simulink model "afe_rst_inv_psm_distributed_control_two_delays"  (R2026a)
settings: Solver=ode1be  StopTime=simlength  FixedStep=tc  MaxStep=Tc
values from neighbouring files (symbols this model uses):
  Amplitude_U = 1.16    [grid_fault_generator.m]
  Amplitude_V = Amplitude_U    (= 1.16)    [grid_fault_generator.m]
  Amplitude_W = Amplitude_U    (= 1.16)    [grid_fault_generator.m]
  end_time_LVRT = start_time_LVRT + error_length    [grid_fault_generator.m]
  Igrid_phase_normalization_factor = 270*sqrt(2)    [grid_emulator.m]
  omega_grid_emulator_nom = w_grid    (= 314.159265359)    [grid_emulator.m]
  omega_grid_nom = w_grid    (= 314.159265359)    [grid_emulator.m]
  t_ramp = 20e-3    (= 0.02)    [grid_fault_generator.m]
  ugrid_factor = 1    [grid_emulator.m]
  V_phase_normalization_factor = Vgrid_phase_normalization_factor    [grid_emulator.m]
  Vdc_bez = 1070    [grid_emulator.m]
  Vemu_ref_norm = Vemu_ref * sqrt(2) / V_phase_normalization_factor    [grid_emulator.m]
  vn_eta_pu = 0    [grid_emulator.m]
  vn_xi_pu = 0    [grid_emulator.m]
  vp_xi_pu = 1    [grid_emulator.m]
undefined symbols (not defined in the file or in its folder): Adrso, Aresd, Bresd, CFi, CFu, Cresd, Crso, CTRPIFF_CLIP_RELEASE, dead_time_INV, emf_fb_p, emf_fb_p_ccaller_1, emf_fb_p_ccaller_2, emf_p, emf_p_ccaller_1, emf_p_ccaller_2, fPWM_INV, g0_161Hz, g0_500Hz, g1_161Hz, g1_500Hz, i_grid_neg_eta_lim, i_grid_neg_eta_red_lim, i_grid_neg_xi_lim, i_grid_neg_xi_red_lim, i_grid_pos_eta_lim, i_grid_pos_eta_red_lim, ibez, id_lim, ieta_neg_ref_lim, ieta_pos_ref_lim, iq_lim, ixi_pos_ref_lim, Jm_norm, k_frt_ref, kg, ki_afe, ki_i, ki_id, ki_iq, ki_rc_neg_grid, ki_rc_pos_grid, ki_vs, ki_w, kp_afe, kp_i, kp_id, kp_iq, kp_rc_neg_grid, kp_rc_pos_grid, kp_vs, kp_w, kw, l1, l2, Lalpha_norm, Ld_norm, Ldrso, Lq_norm, Ls_norm, luenberger_l1 ... (+30)
libraries: fl_lib x146, nesl_utility x62, simulink x8, cstblocks_lti x7, sl_discontinuities x3, single_phase_transformer_lib x3, flexshaft_lib x1, permanent_magnet_synchronous_machine x1
(part 10 of 14)

== system afe_rst_inv_psm_distributed_control_two_delays/INV-Modular/inv_leg_u/driver_board_u/motor_vector_control/bemf_observer/bemf_observer_simulink ==
  ialpha_pu : Inport
  ibeta_pu : Inport  Port=2
  ualpha_pu : Inport  Port=3
  ubeta_pu : Inport  Port=4
  Gain : Gain  Gain=psi_m_norm
  Gain1 : Gain  Gain=psi_m_norm
  Trigonometric Function : Trigonometry  Operator=cos
  Trigonometric Function1 : Trigonometry
  double_integrator_observer : Subsystem
  omega_hat_flt : Subsystem
  psi_alpha_hat : Subsystem
  psi_beta_hat : Subsystem
  theta_bemf_hat : Subsystem
  omega_pu_hat : Outport
  theta_hat : Outport  Port=2
  tag scope: psi_r_m_alpha_dbu=global, psi_r_m_beta_dbu=global, theta_bemf_hat_dbu=global
  wires:
  omega_hat_flt/1(omega_hat_flt) -> theta_bemf_hat/3(omega_pu_hat)
  double_integrator_observer/1(omega_pu_hat) -> omega_hat_flt/1(omega_hat), omega_pu_hat/1  "omega_pu_hat"
  double_integrator_observer/2(theta_hat) -> theta_hat/1  "theta_hat"
  [theta_bemf_hat_dbu] -> double_integrator_observer/1(theta)
  theta_bemf_hat/1(theta_emf_hat) -> [theta_bemf_hat_dbu]
  Gain1/1 -> [psi_r_m_beta_dbu]
  Gain/1 -> [psi_r_m_alpha_dbu]
  [theta_hat_dbu] -> Trigonometric Function1/1, Trigonometric Function/1
  ubeta_pu/1 -> psi_beta_hat/1(ubeta)
  ualpha_pu/1 -> psi_alpha_hat/1(ualpha)
  ibeta_pu/1 -> psi_beta_hat/2(ibeta)
  ialpha_pu/1 -> psi_alpha_hat/2(ialpha)
  Trigonometric Function1/1 -> Gain1/1
  Trigonometric Function/1 -> Gain/1
  [psi_r_alpha_hat_dbu] -> theta_bemf_hat/1(psi_r_alpha_hat)
  [psi_r_beta_hat_dbu] -> theta_bemf_hat/2(psi_r_beta_hat)

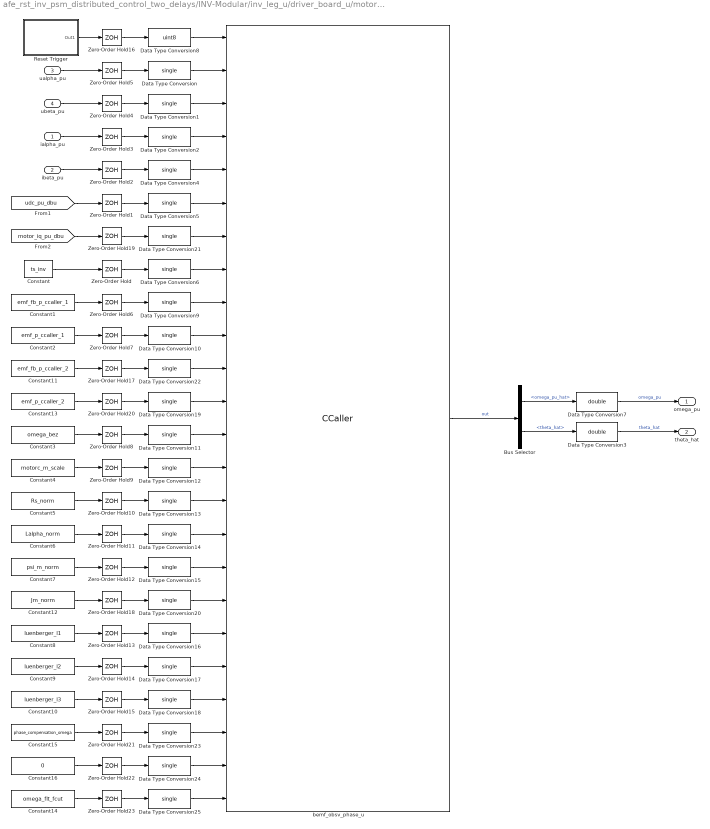
== system afe_rst_inv_psm_distributed_control_two_delays/INV-Modular/inv_leg_u/driver_board_u/motor_vector_control/bemf_observer/bemf_observer_with_load_estimator_ccaller ==
  ialpha_pu : Inport
  ibeta_pu : Inport  Port=2
  ualpha_pu : Inport  Port=3
  ubeta_pu : Inport  Port=4
  Bus Selector : BusSelector  OutputSignals=omega_pu_hat,theta_hat
  Constant : Constant  Value=ts_inv
  Constant1 : Constant  Value=emf_fb_p_ccaller_1
  Constant10 : Constant  Value=luenberger_l3
  Constant11 : Constant  Value=emf_fb_p_ccaller_2
  Constant12 : Constant  Value=Jm_norm
  Constant13 : Constant  Value=emf_p_ccaller_2
  Constant14 : Constant  Value=omega_flt_fcut
  Constant15 : Constant  Value=phase_compensation_omega
  Constant16 : Constant  Value=0
  Constant2 : Constant  Value=emf_p_ccaller_1
  Constant3 : Constant  Value=omega_bez
  Constant4 : Constant  Value=motorc_m_scale
  Constant5 : Constant  Value=Rs_norm
  Constant6 : Constant  Value=Lalpha_norm
  Constant7 : Constant  Value=psi_m_norm
  Constant8 : Constant  Value=luenberger_l1
  Constant9 : Constant  Value=luenberger_l2
  Data Type Conversion{,1..2,4..6,9..25} (23 alike) : DataTypeConversion  OutDataTypeStr=single  SaturateOnIntegerOverflow=off  RndMeth=Floor
  Data Type Conversion3 : DataTypeConversion  OutDataTypeStr=double  SaturateOnIntegerOverflow=off  RndMeth=Floor
  Data Type Conversion7 : DataTypeConversion  OutDataTypeStr=double  SaturateOnIntegerOverflow=off  RndMeth=Floor
  Data Type Conversion8 : DataTypeConversion  OutDataTypeStr=uint8  SaturateOnIntegerOverflow=off  RndMeth=Floor
  Reset Trigger : Subsystem
  Zero-Order Hold{,1..23} (24 alike) : ZeroOrderHold  SampleTime=ts_inv
  bemf_obsv_phase_u : CCaller  FunctionName=bemf_obsv_load_est_process_simulink  PortSpecificationStruct="%)30     .    (\"P   8    (     @         %    \"    !D    !     0         %  0 \"0    $    _    07)G3F%M90  4&]R=$YA;64 4V-O<&4     26YD97@     5'EP90      4VEZ90      27-';&]B86P   X    P    !@    @    $          4    (     0    ,    !         !   P!O=70 #@   #     &    \"     0         !0    @    !     P    $         $  # &]U=  .    .     8    (    !          %    \"     $    &     0         0  ...(+14838 chars)"  SampleTime=ts_inv
  omega_pu : Outport
  theta_hat : Outport  Port=2
  wires:
  Data Type Conversion5/1 -> bemf_obsv_phase_u/6
  Data Type Conversion/1 -> bemf_obsv_phase_u/2
  bemf_obsv_phase_u/1 -> Bus Selector/1  "out"
  Data Type Conversion1/1 -> bemf_obsv_phase_u/3
  Data Type Conversion4/1 -> bemf_obsv_phase_u/5
  Data Type Conversion2/1 -> bemf_obsv_phase_u/4
  Zero-Order Hold/1 -> Data Type Conversion6/1
  Zero-Order Hold5/1 -> Data Type Conversion/1
  Zero-Order Hold4/1 -> Data Type Conversion1/1
  Zero-Order Hold3/1 -> Data Type Conversion2/1
  Zero-Order Hold2/1 -> Data Type Conversion4/1
  Zero-Order Hold1/1 -> Data Type Conversion5/1
  [udc_pu_dbu] -> Zero-Order Hold1/1
  Constant/1 -> Zero-Order Hold/1
  ualpha_pu/1 -> Zero-Order Hold5/1
  ialpha_pu/1 -> Zero-Order Hold3/1
  ubeta_pu/1 -> Zero-Order Hold4/1
  ibeta_pu/1 -> Zero-Order Hold2/1
  Bus Selector/2 -> Data Type Conversion3/1  "<theta_hat>"
  Bus Selector/1 -> Data Type Conversion7/1  "<omega_pu_hat>"
  Data Type Conversion7/1 -> omega_pu/1  "omega_pu"
  Data Type Conversion3/1 -> theta_hat/1  "theta_hat"
  Reset Trigger/1(Out1) -> Zero-Order Hold16/1
  Data Type Conversion8/1 -> bemf_obsv_phase_u/1
  Constant1/1 -> Zero-Order Hold6/1
  Zero-Order Hold6/1 -> Data Type Conversion9/1
  Zero-Order Hold7/1 -> Data Type Conversion10/1
  Zero-Order Hold8/1 -> Data Type Conversion11/1
  Zero-Order Hold9/1 -> Data Type Conversion12/1
  Zero-Order Hold10/1 -> Data Type Conversion13/1
  Zero-Order Hold11/1 -> Data Type Conversion14/1
  Zero-Order Hold12/1 -> Data Type Conversion15/1
  Zero-Order Hold13/1 -> Data Type Conversion16/1
  Zero-Order Hold14/1 -> Data Type Conversion17/1
  Constant2/1 -> Zero-Order Hold7/1
  Constant3/1 -> Zero-Order Hold8/1
  Constant4/1 -> Zero-Order Hold9/1
  Constant5/1 -> Zero-Order Hold10/1
  Constant6/1 -> Zero-Order Hold11/1
  Constant7/1 -> Zero-Order Hold12/1
  Constant8/1 -> Zero-Order Hold13/1
  Constant9/1 -> Zero-Order Hold14/1
  Constant10/1 -> Zero-Order Hold15/1
  Zero-Order Hold15/1 -> Data Type Conversion18/1
  Zero-Order Hold16/1 -> Data Type Conversion8/1
  Constant12/1 -> Zero-Order Hold18/1
  Zero-Order Hold18/1 -> Data Type Conversion20/1
  Data Type Conversion6/1 -> bemf_obsv_phase_u/8
  Data Type Conversion9/1 -> bemf_obsv_phase_u/9
  Data Type Conversion10/1 -> bemf_obsv_phase_u/10
  [motor_iq_pu_dbu] -> Zero-Order Hold19/1
  Zero-Order Hold19/1 -> Data Type Conversion21/1
  Data Type Conversion21/1 -> bemf_obsv_phase_u/7
  Constant13/1 -> Zero-Order Hold20/1
  Zero-Order Hold20/1 -> Data Type Conversion19/1
  Zero-Order Hold17/1 -> Data Type Conversion22/1
  Constant11/1 -> Zero-Order Hold17/1
  Data Type Conversion22/1 -> bemf_obsv_phase_u/11
  Data Type Conversion19/1 -> bemf_obsv_phase_u/12
  Data Type Conversion11/1 -> bemf_obsv_phase_u/13
  Data Type Conversion12/1 -> bemf_obsv_phase_u/14
  Data Type Conversion13/1 -> bemf_obsv_phase_u/15
  Data Type Conversion14/1 -> bemf_obsv_phase_u/16
  Data Type Conversion15/1 -> bemf_obsv_phase_u/17
  Data Type Conversion20/1 -> bemf_obsv_phase_u/18
  Data Type Conversion16/1 -> bemf_obsv_phase_u/19
  Data Type Conversion17/1 -> bemf_obsv_phase_u/20
  Data Type Conversion18/1 -> bemf_obsv_phase_u/21
  Zero-Order Hold23/1 -> Data Type Conversion25/1
  Constant14/1 -> Zero-Order Hold23/1
  Constant16/1 -> Zero-Order Hold22/1
  Constant15/1 -> Zero-Order Hold21/1
  Zero-Order Hold22/1 -> Data Type Conversion24/1
  Zero-Order Hold21/1 -> Data Type Conversion23/1
  Data Type Conversion23/1 -> bemf_obsv_phase_u/22
  Data Type Conversion24/1 -> bemf_obsv_phase_u/23
  Data Type Conversion25/1 -> bemf_obsv_phase_u/24

== system afe_rst_inv_psm_distributed_control_two_delays/INV-Modular/inv_leg_u/driver_board_u/motor_vector_control/current_ctrl/MTPA ==
  iq : Inport
  Constant : Constant  Value=psi_m_norm
  Gain1 : Gain  Gain=1/(Lq_norm - Ld_norm)/2
  Gain2 : Gain  Gain=1/(Lq_norm - Ld_norm)/2
  Math Function1 : Math  Operator=magnitude^2  SignedPower=on
  Math Function4 : Math  Operator=magnitude^2  SignedPower=on
  Sqrt : Sqrt
  Sum : Sum  Inputs=|++
  Sum1 : Sum  Inputs=|+-
  id_ref_pu < x < 0 : Saturate  UpperLimit=0  LowerLimit=-id_lim
  Id_ref_mtpa : Outport  VectorParamsAs1DForOutWhenUnconnected=off
  wires:
  id_ref_pu < x < 0/1 -> Id_ref_mtpa/1
  Gain1/1 -> Math Function4/1
  Math Function1/1 -> Sum/2
  Sum/1 -> Sqrt/1
  Sqrt/1 -> Sum1/2
  iq/1 -> Math Function1/1
  Gain2/1 -> Sum1/1
  Constant/1 -> Gain1/1, Gain2/1
  Sum1/1 -> id_ref_pu < x < 0/1
  Math Function4/1 -> Sum/1

== system afe_rst_inv_psm_distributed_control_two_delays/INV-Modular/inv_leg_u/driver_board_u/motor_vector_control/current_ctrl/dq_pi_with_vector_antiwindup ==
  id_ref : Inport
  id : Inport  Port=2
  iq_ref : Inport  Port=3
  iq : Inport  Port=4
  dq_vector_pi : Subsystem
  dq_vector_pi_ccaller : Subsystem  Commented=on
  ctrl_d_u : Outport
  ctrl_q_u : Outport  Port=2
  wires:
  id/1 -> dq_vector_pi/1(id)  "id"
  id_ref/1 -> dq_vector_pi/2(id_ref)  "id_ref"
  iq/1 -> dq_vector_pi/3(iq)  "iq"
  iq_ref/1 -> dq_vector_pi/4(iq_ref)  "iq_ref"
  dq_vector_pi/1(ctrl_d_u) -> ctrl_d_u/1
  dq_vector_pi/2(ctrl_q_u) -> ctrl_q_u/1

== system afe_rst_inv_psm_distributed_control_two_delays/INV-Modular/inv_leg_u/driver_board_u/motor_vector_control/current_ctrl/id_ref ==
  id_mtpa : Inport
  Constant : Constant  Value=0
  Manual Switch : ManualSwitch
  id_ref : Outport
  wires:
  Manual Switch/1 -> id_ref/1
  id_mtpa/1 -> Manual Switch/1
  Constant/1 -> Manual Switch/2

== system afe_rst_inv_psm_distributed_control_two_delays/INV-Modular/inv_leg_u/modulator/sv_pwm/modulator/PWM generator ==
  m_index : Inport
  Constant : Constant  Value=dead_time*f
  Constant1 : Constant
  Data Type Conversion1 : DataTypeConversion
  Data Type Conversion2 : DataTypeConversion
  Gain : Gain  Gain=1/(pi/2)
  Gain1 : Gain  Gain=1/2
  Gain2 : Gain  Gain=vg_firing
  Gain3 : Gain  Gain=vg_firing
  Gain4 : Gain  Gain=polarity
  Gain5 : Gain  Gain=polarity
  Hit Crossing : HitCross  Commented=on  ShowOutputPort=off
  Hit Crossing1 : HitCross  Commented=on  ShowOutputPort=off
  Relational Operator1 : RelationalOperator  Operator=<=  InputSameDT=off
  Relational Operator2 : RelationalOperator  Operator=<=  InputSameDT=off
  Saturation1 : Saturate  UpperLimit=m_up  LowerLimit=m_low
  Sine Wave : Sin  Frequency=f*2*pi  Phase=-pi/2+ph  SampleTime=0
  Sum : Sum  Inputs=|++  SaturateOnIntegerOverflow=on
  Sum1 : Sum  Inputs=-+|  SaturateOnIntegerOverflow=on
  Sum2 : Sum  Inputs=|++
  Trigonometric Function1 : Trigonometry  Operator=asin
  m1 : Outport
  m2 : Outport  Port=2
  wires:
  Gain5/1 -> m2/1
  Gain4/1 -> m1/1
  Gain3/1 -> Gain5/1
  Gain2/1 -> Gain4/1
  Data Type Conversion1/1 -> Gain2/1, Hit Crossing/1
  Gain1/1 -> Relational Operator1/2, Relational Operator2/1
  Sum2/1 -> Gain1/1
  Gain/1 -> Sum2/1
  Trigonometric Function1/1 -> Gain/1
  Constant1/1 -> Sum2/2
  Sine Wave/1 -> Trigonometric Function1/1
  Sum1/1 -> Relational Operator2/2
  Sum/1 -> Relational Operator1/1
  Saturation1/1 -> Sum1/2, Sum/1
  Constant/1 -> Sum1/1, Sum/2
  Data Type Conversion2/1 -> Hit Crossing1/1, Gain3/1
  Relational Operator2/1 -> Data Type Conversion2/1
  m_index/1 -> Saturation1/1
  Relational Operator1/1 -> Data Type Conversion1/1

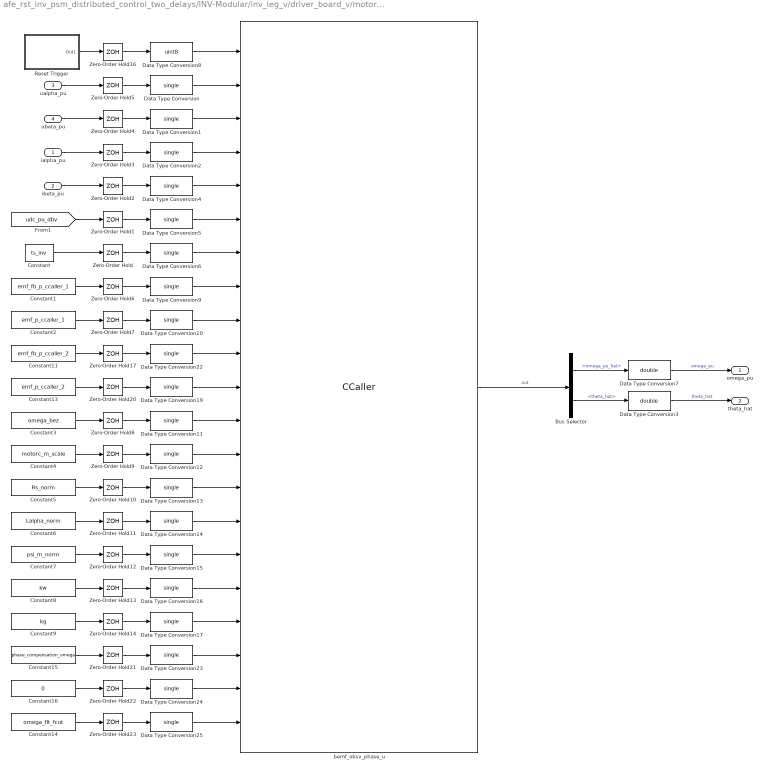
== system afe_rst_inv_psm_distributed_control_two_delays/INV-Modular/inv_leg_v/driver_board_v/motor_vector_control/bemf_observer/bemf_observer_ccaller ==
  ialpha_pu : Inport
  ibeta_pu : Inport  Port=2
  ualpha_pu : Inport  Port=3
  ubeta_pu : Inport  Port=4
  Bus Selector : BusSelector  OutputSignals=omega_pu_hat,theta_hat
  Constant : Constant  Value=ts_inv
  Constant1 : Constant  Value=emf_fb_p_ccaller_1
  Constant11 : Constant  Value=emf_fb_p_ccaller_2
  Constant13 : Constant  Value=emf_p_ccaller_2
  Constant14 : Constant  Value=omega_flt_fcut
  Constant15 : Constant  Value=phase_compensation_omega
  Constant16 : Constant  Value=0
  Constant2 : Constant  Value=emf_p_ccaller_1
  Constant3 : Constant  Value=omega_bez
  Constant4 : Constant  Value=motorc_m_scale
  Constant5 : Constant  Value=Rs_norm
  Constant6 : Constant  Value=Lalpha_norm
  Constant7 : Constant  Value=psi_m_norm
  Constant8 : Constant  Value=kw
  Constant9 : Constant  Value=kg
  Data Type Conversion{,1..2,4..6,9..17,19,22..25} (20 alike) : DataTypeConversion  OutDataTypeStr=single  SaturateOnIntegerOverflow=off  RndMeth=Floor
  Data Type Conversion3 : DataTypeConversion  OutDataTypeStr=double  SaturateOnIntegerOverflow=off  RndMeth=Floor
  Data Type Conversion7 : DataTypeConversion  OutDataTypeStr=double  SaturateOnIntegerOverflow=off  RndMeth=Floor
  Data Type Conversion8 : DataTypeConversion  OutDataTypeStr=uint8  SaturateOnIntegerOverflow=off  RndMeth=Floor
  Reset Trigger : Subsystem
  Zero-Order Hold{,1..14,16..17,20..23} (21 alike) : ZeroOrderHold  SampleTime=ts_inv
  bemf_obsv_phase_u : CCaller  FunctionName=bemf_obsv_process_simulink  PortSpecificationStruct="%)30     .    N\"8   8    (     @         %    \"    !8    !     0         %  0 \"0    $    _    07)G3F%M90  4&]R=$YA;64 4V-O<&4     26YD97@     5'EP90      4VEZ90      27-';&]B86P   X    P    !@    @    $          4    (     0    ,    !         !   P!O=70 #@   #     &    \"     0         !0    @    !     P    $         $  # &]U=  .    .     8    (    !          %    \"     $    &     0         0  ...(+12985 chars)"  SampleTime=ts_inv
  omega_pu : Outport
  theta_hat : Outport  Port=2
  wires:
  Zero-Order Hold21/1 -> Data Type Conversion23/1
  Zero-Order Hold22/1 -> Data Type Conversion24/1
  Constant15/1 -> Zero-Order Hold21/1
  Constant16/1 -> Zero-Order Hold22/1
  Constant14/1 -> Zero-Order Hold23/1
  Zero-Order Hold23/1 -> Data Type Conversion25/1
  Constant11/1 -> Zero-Order Hold17/1
  Zero-Order Hold17/1 -> Data Type Conversion22/1
  Zero-Order Hold20/1 -> Data Type Conversion19/1
  Constant13/1 -> Zero-Order Hold20/1
  Zero-Order Hold16/1 -> Data Type Conversion8/1
  Constant9/1 -> Zero-Order Hold14/1
  Constant8/1 -> Zero-Order Hold13/1
  Constant7/1 -> Zero-Order Hold12/1
  Constant6/1 -> Zero-Order Hold11/1
  Constant5/1 -> Zero-Order Hold10/1
  Constant4/1 -> Zero-Order Hold9/1
  Constant3/1 -> Zero-Order Hold8/1
  Constant2/1 -> Zero-Order Hold7/1
  Zero-Order Hold14/1 -> Data Type Conversion17/1
  Zero-Order Hold13/1 -> Data Type Conversion16/1
  Zero-Order Hold12/1 -> Data Type Conversion15/1
  Zero-Order Hold11/1 -> Data Type Conversion14/1
  Zero-Order Hold10/1 -> Data Type Conversion13/1
  Zero-Order Hold9/1 -> Data Type Conversion12/1
  Zero-Order Hold8/1 -> Data Type Conversion11/1
  Zero-Order Hold7/1 -> Data Type Conversion10/1
  Zero-Order Hold6/1 -> Data Type Conversion9/1
  Constant1/1 -> Zero-Order Hold6/1
  Data Type Conversion8/1 -> bemf_obsv_phase_u/1
  Reset Trigger/1(Out1) -> Zero-Order Hold16/1
  Data Type Conversion3/1 -> theta_hat/1  "theta_hat"
  Data Type Conversion7/1 -> omega_pu/1  "omega_pu"
  Bus Selector/1 -> Data Type Conversion7/1  "<omega_pu_hat>"
  Bus Selector/2 -> Data Type Conversion3/1  "<theta_hat>"
  ibeta_pu/1 -> Zero-Order Hold2/1
  ubeta_pu/1 -> Zero-Order Hold4/1
  ialpha_pu/1 -> Zero-Order Hold3/1
  ualpha_pu/1 -> Zero-Order Hold5/1
  Constant/1 -> Zero-Order Hold/1
  [udc_pu_dbv] -> Zero-Order Hold1/1
  Zero-Order Hold1/1 -> Data Type Conversion5/1
  Zero-Order Hold2/1 -> Data Type Conversion4/1
  Zero-Order Hold3/1 -> Data Type Conversion2/1
  Zero-Order Hold4/1 -> Data Type Conversion1/1
  Zero-Order Hold5/1 -> Data Type Conversion/1
  Zero-Order Hold/1 -> Data Type Conversion6/1
  Data Type Conversion2/1 -> bemf_obsv_phase_u/4
  Data Type Conversion4/1 -> bemf_obsv_phase_u/5
  Data Type Conversion1/1 -> bemf_obsv_phase_u/3
  bemf_obsv_phase_u/1 -> Bus Selector/1  "out"
  Data Type Conversion/1 -> bemf_obsv_phase_u/2
  Data Type Conversion5/1 -> bemf_obsv_phase_u/6
  Data Type Conversion23/1 -> bemf_obsv_phase_u/19
  Data Type Conversion24/1 -> bemf_obsv_phase_u/20
  Data Type Conversion25/1 -> bemf_obsv_phase_u/21
  Data Type Conversion17/1 -> bemf_obsv_phase_u/18
  Data Type Conversion16/1 -> bemf_obsv_phase_u/17
  Data Type Conversion15/1 -> bemf_obsv_phase_u/16
  Data Type Conversion14/1 -> bemf_obsv_phase_u/15
  Data Type Conversion13/1 -> bemf_obsv_phase_u/14
  Data Type Conversion12/1 -> bemf_obsv_phase_u/13
  Data Type Conversion11/1 -> bemf_obsv_phase_u/12
  Data Type Conversion19/1 -> bemf_obsv_phase_u/11
  Data Type Conversion22/1 -> bemf_obsv_phase_u/10
  Data Type Conversion10/1 -> bemf_obsv_phase_u/9
  Data Type Conversion9/1 -> bemf_obsv_phase_u/8
  Data Type Conversion6/1 -> bemf_obsv_phase_u/7

== system afe_rst_inv_psm_distributed_control_two_delays/INV-Modular/inv_leg_v/driver_board_v/motor_vector_control/bemf_observer/bemf_observer_simulink ==
  ialpha_pu : Inport
  ibeta_pu : Inport  Port=2
  ualpha_pu : Inport  Port=3
  ubeta_pu : Inport  Port=4
  Gain : Gain  Gain=psi_m_norm
  Gain1 : Gain  Gain=psi_m_norm
  Trigonometric Function : Trigonometry  Operator=cos
  Trigonometric Function1 : Trigonometry
  double_integrator_observer : Subsystem
  omega_hat_flt : Subsystem
  psi_alpha_hat : Subsystem
  psi_beta_hat : Subsystem
  theta_bemf_hat : Subsystem
  omega_pu_hat : Outport
  theta_hat : Outport  Port=2
  tag scope: psi_r_m_alpha_dbv=global, psi_r_m_beta_dbv=global, theta_bemf_hat_dbv=global
  wires:
  omega_hat_flt/1(omega_hat_flt) -> theta_bemf_hat/3(omega_pu_hat)
  double_integrator_observer/1(omega_pu_hat) -> omega_hat_flt/1(omega_hat), omega_pu_hat/1  "omega_pu_hat"
  double_integrator_observer/2(theta_hat) -> theta_hat/1  "theta_hat"
  [theta_bemf_hat_dbv] -> double_integrator_observer/1(theta)
  theta_bemf_hat/1(theta_emf_hat) -> [theta_bemf_hat_dbv]
  Gain1/1 -> [psi_r_m_beta_dbv]
  Gain/1 -> [psi_r_m_alpha_dbv]
  [theta_hat_dbv] -> Trigonometric Function1/1, Trigonometric Function/1
  ubeta_pu/1 -> psi_beta_hat/1(ubeta)
  ualpha_pu/1 -> psi_alpha_hat/1(ualpha)
  ibeta_pu/1 -> psi_beta_hat/2(ibeta)
  ialpha_pu/1 -> psi_alpha_hat/2(ialpha)
  Trigonometric Function1/1 -> Gain1/1
  Trigonometric Function/1 -> Gain/1
  [psi_r_alpha_hat_dbv] -> theta_bemf_hat/1(psi_r_alpha_hat)
  [psi_r_beta_hat_dbv] -> theta_bemf_hat/2(psi_r_beta_hat)
